simulink model "ev_powertrain"  (R2025b)
settings: Solver=ode45  StartTime=0.0  StopTime=p.stopTime  MaxStep=p.sampleTime  RelTol=1e-8  AbsTol=1e-10
model workspace (MAT data in the model file):
  inputSignal = [0 0.02 0.04 0.06 0.08 0.1 0.1 0.12 0.14 0.16 0.18 0.2 ... (16205 elements, 3241x5)]
  p.mass = 1600
  p.gravity = 9.81
  p.rollingCoefficient = 0.01
  p.dragArea = 0.6
  p.airDensity = 1.2
  p.wheelRadius = 0.31
  p.gearRatio = 9
  p.gearEfficiency = 0.97
  p.peakTorque = 310
  p.peakPower = 150000
  p.maximumMotorSpeed = 1500
  p.motorTimeConstant = 0.07
  p.capacityAh = 166.666666667
  p.batteryResistance = 0.08
  p.auxiliaryPower = 400
  p.usableEnergy_kWh = 54
  p.driverKp = 900
  p.driverKi = 250
  p.driverTracking = 2
  p.citySpeed = 15
  p.fastSpeed = 25
  p.rampStart = 0.1
  p.accelerationDuration = 4
  p.brakeDuration = 8
  p.grade = 0.03
  p.gradeTime = 14.08
  p.fastTime = 26.34
  p.flatTime = 44
  p.brakeTime = 56.32
  p.sampleTime = 0.02
  p.sizingDuration = 20
  p.stopTime = 64.64
  p.regenMode = 1
  p.initialState = [0; 0; 0.8; 0; 0; 0; 0]
  p.initialControlState = 0
  p.modelName = 'ev_powertrain'
values from neighbouring files (symbols this model uses):
  p = project_parameters();[p,timing]=plan_experiment(p)    [run_demo.m]
undefined symbols (not defined in the file or in its folder): sl_controller, sl_plant
settings Model: Creator=LENOVO  LastModifiedBy=LENOVO

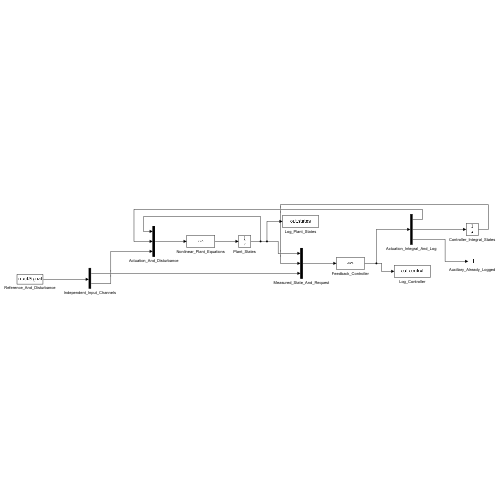
[thumbnail: Simulink's stored preview of the top-level diagram]
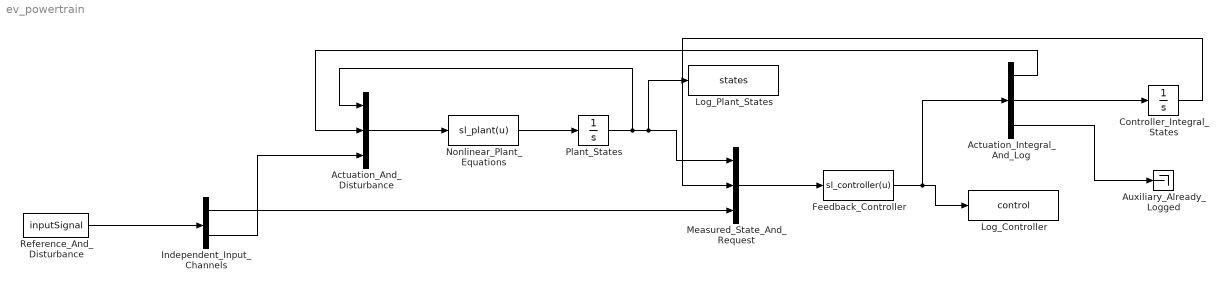
== system ev_powertrain ==
  Actuation_And_Disturbance : Mux  Inputs=3
  Actuation_Integral_And_Log : Demux  Outputs=[2 1 3]
  Auxiliary_Already_Logged : Terminator
  Controller_Integral_States : Integrator  InitialCondition=p.initialControlState
  Feedback_Controller : MATLABFcn  MATLABFcn=sl_controller(u)  OutputDimensions=6
  Independent_Input_Channels : Demux  Outputs=[3 1]
  Log_Controller : ToWorkspace  VariableName=control  SaveFormat=Timeseries  SampleTime=-1
  Log_Plant_States : ToWorkspace  VariableName=states  SaveFormat=Timeseries  SampleTime=-1
  Measured_State_And_Request : Mux  Inputs=3
  Nonlinear_Plant_Equations : MATLABFcn  MATLABFcn=sl_plant(u)  OutputDimensions=7
  Plant_States : Integrator  InitialCondition=p.initialState
  Reference_And_Disturbance : FromWorkspace  VariableName=inputSignal  OutputAfterFinalValue=Holding final value
  wires:
  Nonlinear_Plant_Equations/1 -> Plant_States/1
  Actuation_And_Disturbance/1 -> Nonlinear_Plant_Equations/1
  Independent_Input_Channels/2 -> Actuation_And_Disturbance/3
  Actuation_Integral_And_Log/1 -> Actuation_And_Disturbance/2
  Actuation_Integral_And_Log/3 -> Auxiliary_Already_Logged/1
  Actuation_Integral_And_Log/2 -> Controller_Integral_States/1
  Feedback_Controller/1 -> Actuation_Integral_And_Log/1, Log_Controller/1
  Measured_State_And_Request/1 -> Feedback_Controller/1
  Independent_Input_Channels/1 -> Measured_State_And_Request/3
  Controller_Integral_States/1 -> Measured_State_And_Request/2
  Plant_States/1 -> Measured_State_And_Request/1, Log_Plant_States/1, Actuation_And_Disturbance/1
  Reference_And_Disturbance/1 -> Independent_Input_Channels/1
